simulink model "Sim2Real_ankle_motion_2025a"  (R2025a)
settings: Solver=FixedStepDiscrete  StartTime=0.0  StopTime=8  FixedStep=Ts_1ms  MaxStep=0.002  RelTol=1e-3
InitFcn:
  | modelFile = get_param(bdroot,'FileName');
  | if isempty(modelFile)
  |     error('The model must be saved before running InitFcn.');
  | end
  | 
  | % Folder where the .slx model is located
  | modelFolder = fileparts(char(modelFile));
  | 
  | % Find the parent folder named "resources" by going upwards
  | currentFolder  = modelFolder;
  | materialFolder = '';
  | 
  | while true
  |     [parentFolder, currentName] = fileparts(currentFolder);
  | 
  |     if strcmpi(currentName, 'resources')
  |         materialFolder = currentFolder;
  |         break;
  |     end
  | 
  |     if strcmp(parentFolder, currentFolder)
  |         error('Could not find a parent folder named "resources" starting from: %s', modelFolder);
  |     end
  | 
  |     currentFolder = parentFolder;
  | end
  | 
  | % Search recursively for the MuJoCo XML inside "material"
  | xmlSearch = dir(fullfile(materialFolder, '**', 'unitree_G1.xml'));
  | 
  | if isempty(xmlSearch)
  |     error('MuJoCo XML file not found inside material folder: %s', materialFolder);
  | elseif numel(xmlSearch) > 1
  |     error('Multiple unitree_G1.xml files found inside material folder. Leave only one valid XML.');
  | end
  | 
  | mujocoFolder = xmlSearch(1).folder;
  | xmlFullPath  = fullfile(xmlSearch(1).folder, xmlSearch(1).name);
  | 
  | % Save in base workspace in case you want to inspect them
  | assignin('base','modelFolder',modelFolder);
  | assignin('base','materialFolder',materialFolder);
  | assignin('base','mujocoFolder',mujocoFolder);
  | assignin('base','xmlFullPath',xmlFullPath);
  | 
  | % Final existence check
  | if exist(xmlFullPath,'file') ~= 2
  |     error('MuJoCo XML file not found: %s', xmlFullPath);
  | end
  | 
  | % Add the XML folder to the path so WHICH can find it
  | addpath(mujocoFolder, '-begin');
  | rehash path;
  | 
  | % Run launcher from the same folder as the model
  | launcherFile = fullfile(modelFolder, 'launcher_ankle_motion.mlx');
  | if exist(launcherFile,'file') == 2
  |     run(launcherFile);
  | else
  |     error('Launcher file not found: %s', launcherFile);
  | end
  | 
  | % RUN_MODE:
  | if evalin('base', "exist('RUN_MODE','var')")
  |     tmp = evalin('base','RUN_MODE');
  |     if isa(tmp,'Simulink.Parameter')
  |         RUN_MODE = tmp;
  |     else
  |         RUN_MODE = Simulink.Parameter(tmp);
  |         RUN_MODE.CoderInfo.StorageClass = 'SimulinkGlobal';
  |         assignin('base','RUN_MODE',RUN_MODE);
  |     end
  | else
  |     RUN_MODE = Simulink.Parameter(0);
  |     RUN_MODE.CoderInfo.StorageClass = 'SimulinkGlobal';
  |     assignin('base','RUN_MODE',RUN_MODE);
  | end
StopFcn:
  | drawnow; pause(0.05);
  | 
  | % Stop figures
  | tags = {'G1_IMUState','G1_MotorState'};
  | for k = 1:numel(tags)
  |     delete(findall(0,'Type','uifigure','Tag',tags{k}));
  |     delete(findall(0,'Type','figure' , 'Tag',tags{k}));
  | end
  | 
  | 
  | % Automatic ankle metrics CSV (installed once)
  | addpath(fileparts(get_param('Sim2Real_ankle_motion_2025a', 'FileName')));
  | ankle_motion_csv('save');
undefined symbols (not defined in the file or in its folder): crc, DiscIntNeverNeededParam, mode_machine, mode_pr, motor_cmd, reserve, Ts_1ms
libraries: ros2lib x3, slpidlib x1, mjLib x1
(part 1 of 2)
settings Model: Creator=vmano  LastModifiedBy=Leffer
settings OptimizationCC: ReuseModelBlockBuffer=off
settings ModelReferenceCC: EnableRefExpFcnMdlSchedulingChecks=on
settings SFSimCC: SimTargetLang=C++  SimDLTargetLibrary=mkl-dnn
settings RTWCC: GPUComputeCapability=3.5

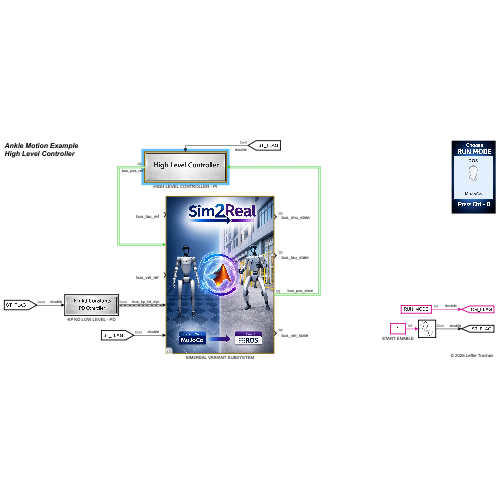
[thumbnail: Simulink's stored preview of the top-level diagram]
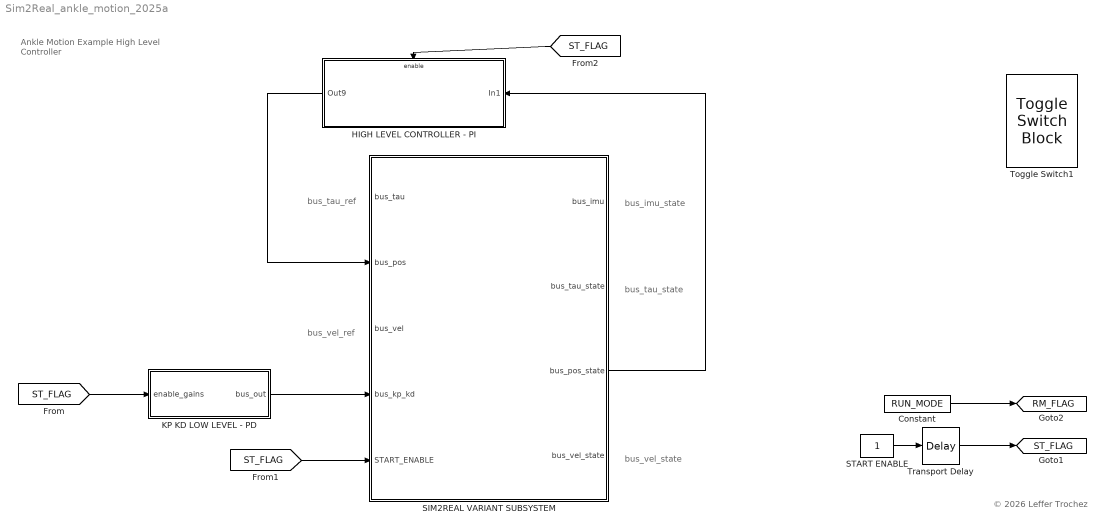
== system Sim2Real_ankle_motion_2025a ==
  note: bus_tau_ref
  note: © 2026 Leffer Trochez
  note: bus_vel_ref
  note: bus_imu_state
  note: bus_tau_state
  note: bus_vel_state
  note: Ankle Motion Example
      | High Level Controller
  Constant : Constant  Value=RUN_MODE
  HIGH LEVEL CONTROLLER - PI : Subsystem  TreatAsAtomicUnit=on
      mask Display: image('16.png');
  KP KD LOW LEVEL - PD : MATLAB Function  TreatAsAtomicUnit=on
  SIM2REAL VARIANT SUBSYSTEM : Subsystem  Variant=on  EmptyChoice=on
      mask Display: image('Sim2RealLogo2.png');
  START ENABLE : Constant
  Toggle Switch1 : ToggleSwitchBlock  LabelPosition=Hide
  Transport Delay : TransportDelay  DelayTime=3  BufferSize=8192
  tag scope: RM_FLAG=global, ST_FLAG=global
  wires:
  Constant/1 -> [RM_FLAG]
  KP KD LOW LEVEL - PD/1(bus_out) -> SIM2REAL VARIANT SUBSYSTEM/4(bus_kp_kd)
  START ENABLE/1 -> Transport Delay/1
  Transport Delay/1 -> [ST_FLAG]
  [ST_FLAG] -> KP KD LOW LEVEL - PD/1(enable_gains)
  [ST_FLAG] -> SIM2REAL VARIANT SUBSYSTEM/5(START_ENABLE)
  SIM2REAL VARIANT SUBSYSTEM/3(bus_pos_state) -> HIGH LEVEL CONTROLLER - PI/1(In1)
  HIGH LEVEL CONTROLLER - PI/1(Out9) -> SIM2REAL VARIANT SUBSYSTEM/2(bus_pos)
  [ST_FLAG] -> HIGH LEVEL CONTROLLER - PI/Enable

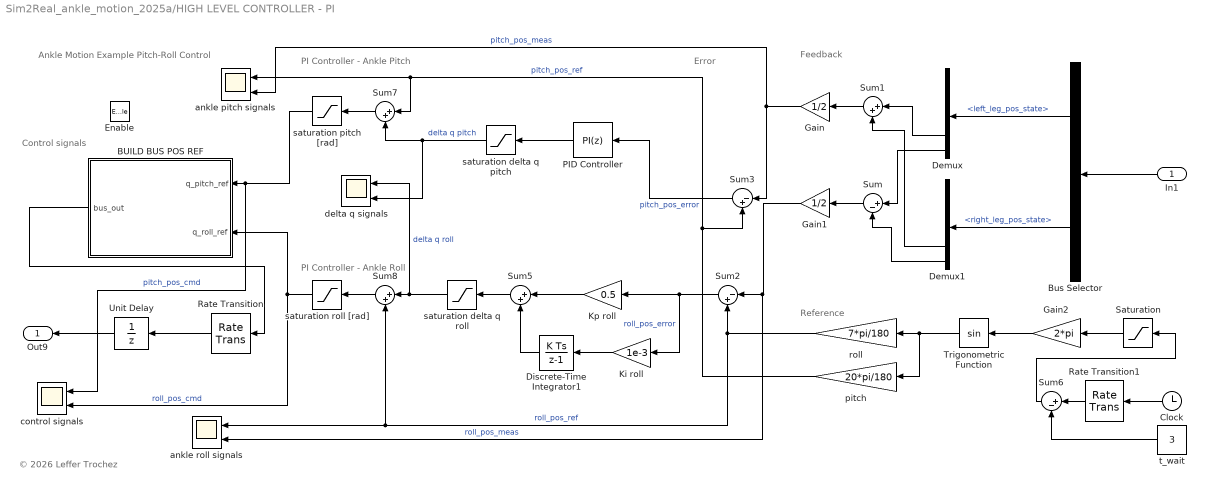
== system Sim2Real_ankle_motion_2025a/HIGH LEVEL CONTROLLER - PI ==
  note: Ankle Motion Example
      | Pitch-Roll Control
  note: Reference
  note: Feedback
  note: PI Controller - Ankle Pitch
  note: PI Controller - Ankle Roll
  note: Error
  note: Control signals
  note: © 2026 Leffer Trochez
  In1 : Inport  OutDataTypeStr=Bus: bus_pos_state
  Enable : EnablePort
  BUILD BUS POS REF : MATLAB Function  TreatAsAtomicUnit=on
  Bus Selector : BusSelector  OutputSignals=left_leg_pos_state,right_leg_pos_state
  Clock : Clock
  Demux : Demux  Outputs=6
  Demux1 : Demux  Outputs=6
  Discrete-Time Integrator1 : DiscreteIntegrator  SampleTime=0.002  ICPrevOutput=DiscIntNeverNeededParam  ICPrevScaledInput=DiscIntNeverNeededParam
  Gain : Gain  Gain=1/2
  Gain1 : Gain  Gain=1/2
  Gain2 : Gain  Gain=2*pi
  Ki roll : Gain  Gain=1e-3
  Kp roll : Gain  Gain=0.5
  "PID Controller " : slpidlib/PID Controller  Controller=PI  Form=Parallel  TimeDomain=Discrete-time  UseExternalTs=off  SampleTime=0.002  IntegratorMethod=Forward Euler  FilterMethod=Forward Euler  ControllerParametersSource=internal  P=0.3  I=0.04  UseKiTs=off  D=0  UseExternalDerivativeSource=off  N=100  UseFilter=on  TunerSelectOption=Transfer Function Based (PID Tuner App)  InitialConditionSource=internal  InitialConditionForIntegrator=0  InitialConditionForFilter=0  DifferentiatorICPrevScaledInput=0  ExternalReset=none  TrackingMode=off  Kt=1  LimitOutput=on  SatLimitsSource=internal  UpperSaturationLimit=0.035  LowerSaturationLimit=-0.035  LinearizeAsGain=on  AntiWindupMode=clamping  Kb=1  LimitIntegrator=off  UpperIntegratorSaturationLimit=inf  LowerIntegratorSaturationLimit=-inf  POutMin=[]  POutMax=[]  IOutMin=[]  IOutMax=[]  DOutMin=[]  DOutMax=[]  NOutMin=[]  NOutMax=[]  SumOutMin=[]  SumOutMax=[]  SaturationOutMin=[]  SaturationOutMax=[]  PParamMin=[]  PParamMax=[]  IParamMin=[]  IParamMax=[]  DParamMin=[]  DParamMax=[]  NParamMin=[]  NParamMax=[]  KbParamMin=[]  KbParamMax=[]  KtParamMin=[]  KtParamMax=[]  KbOutMin=[]  KbOutMax=[]  KtOutMin=[]  KtOutMax=[]  IntegratorOutMin=[]  IntegratorOutMax=[]  FilterOutMin=[]  FilterOutMax=[]  SumI1OutMin=[]  SumI1OutMax=[]  SumI2OutMin=[]  SumI2OutMax=[]  SumI3OutMin=[]  SumI3OutMax=[]  SumI4OutMin=[]  SumI4OutMax=[]  SumDOutMin=[]  SumDOutMax=[]  DifferentiatorOutMin=[]  DifferentiatorOutMax=[]  FilterDiffOutCoefMin=[]  FilterDiffOutCoefMax=[]  ReciprocalOutMin=[]  ReciprocalOutMax=[]  SumDenOutMin=[]  SumDenOutMax=[]  SumNumOutMin=[]  SumNumOutMax=[]  DivideOutMin=[]  DivideOutMax=[]  UdiffTsProdOutMin=[]  UdiffTsProdOutMax=[]  NTsProdOutMin=[]  NTsProdOutMax=[]  UintegralTsProdOutMin=[]  UintegralTsProdOutMax=[]  UngainTsProdOutMin=[]  UngainTsProdOutMax=[]  ClampingZeroOutDataTypeStr=Inherit: Inherit via back propagation  ClampingZeroOutMin=[]  ClampingZeroOutMax=[]  FilterDenConstantOutDataTypeStr=Inherit: Inherit via back propagation  FilterDenConstantOutMin=[]  FilterDenConstantOutMax=[]  PCopyOutDataTypeStr=Inherit: Inherit via back propagation  PCopyOutMin=[]  PCopyOutMax=[]  NCopyOutDataTypeStr=Inherit: Inherit via back propagation  NCopyOutMin=[]  NCopyOutMax=[]  IntegratorContinuousStateAttributes=''  IntegratorStateMustResolveToSignalObject=off  IntegratorRTWStateStorageClass=Auto  FilterContinuousStateAttributes=''  FilterStateMustResolveToSignalObject=off  FilterRTWStateStorageClass=Auto  ParallelPVariant=InternalParameters  IdealPVariant=Disabled  IVariant=InternalParameters  DVariant=Disabled  IntegratorVariant=Discrete  SatVariant=Enabled  AWVariant=DiscClampingParallel  PCopyVariant=Disabled  TRVariant=Disabled  FdbkBlocksVariant=Forward  IdealPFdbkVariant=Disabled  SatFdbkVariant=Disabled  DerivativeFilterVariant=Disabled  NVariant=Disabled  NCopyVariant=Disabled_SignalSpec  FilterICVariant=Disabled  IntegratorICVariant=InternalICs  ExternalResetVariant=Disabled  TRSumVariant=Passthrough  SumFdbkVariant=Disabled  SumVariant=Sum_PI  TsampFilterVariant=InternalTs  TsampNgainVariant=Passthrough  TsampIntegralVariant=Disabled_SignalSpec  ExternalSaturationOutDataTypeStr=Inherit: Same as second input  DerivativeSourceVariant=Disabled  PreIntVariant=InternalPreInt
      settings: LibrarySourceBlock=simulink/Discrete/Discrete PID Controller
  Rate Transition : RateTransition  OutPortSampleTime=Ts_2ms
  Rate Transition1 : RateTransition  OutPortSampleTime=Ts_2ms
  Saturation : Saturate  UpperLimit=inf  LowerLimit=0
  Sum : Sum  Inputs=|+-
  Sum{1,5,7..8} (4 alike) : Sum  Inputs=|++
  Sum2 : Sum  Inputs=|-+
  Sum3 : Sum  Inputs=|-+
  Sum6 : Sum  Inputs=|+-
  Trigonometric Function : Trigonometry
  Unit Delay : UnitDelay  SampleTime=-1  HasFrameUpgradeWarning=on
  ankle pitch signals : Scope  NumInputPorts=2
      settings: Title=Ankle Pitch Signals  ActiveDisplayYMinimum=-0.43633231299858238  ActiveDisplayYMaximum=0.43633231299858238  YLabel=Position [rad]
  ankle roll signals : Scope  NumInputPorts=2
      settings: Title=Ankle Roll Signals  ActiveDisplayYMinimum=-0.15271630954950383  ActiveDisplayYMaximum=0.15271630954950383  YLabel=Position [rad]
  control signals : Scope  NumInputPorts=2
      settings: Title=Torque Position Signals  ActiveDisplayYMinimum=-0.4451715502441761  ActiveDisplayYMaximum=0.44153028177818288  YLabel=Position [rad]  DataLoggingVariableName=ScopeData2
  delta q signals : Scope  NumInputPorts=2
      settings: Title=Delta q Signals  ActiveDisplayYMinimum=-0.0436472558403566  ActiveDisplayYMaximum=0.04282530256320935  DataLoggingVariableName=ScopeData3
  pitch : Gain  Gain=20*pi/180
  roll : Gain  Gain=7*pi/180
  saturation delta q pitch : Saturate  UpperLimit=0.035  LowerLimit=-0.035
  saturation delta q roll : Saturate  UpperLimit=0.025  LowerLimit=-0.025
  saturation pitch [rad] : Saturate  UpperLimit=0.535  LowerLimit=-0.535
  saturation roll [rad] : Saturate  UpperLimit=0.25  LowerLimit=-0.25
  t_wait : Constant  Value=3
  Out9 : Outport  OutDataTypeStr=Bus: bus_pos_ref
  wires:
  Bus Selector/1 -> Demux/1  "<left_leg_pos_state>"
  saturation delta q pitch/1 -> delta q signals/2, Sum7/2  "delta q pitch"
  Gain2/1 -> Trigonometric Function/1
  Rate Transition/1 -> Unit Delay/1
  Sum/1 -> Gain1/1
  "PID Controller "/1 -> saturation delta q pitch/1
  Unit Delay/1 -> Out9/1
  Demux1/6 -> Sum/2
  Kp roll/1 -> Sum5/1
  Sum1/1 -> Gain/1
  Demux1/5 -> Sum1/2
  Discrete-Time Integrator1/1 -> Sum5/2
  Bus Selector/2 -> Demux1/1  "<right_leg_pos_state>"
  Gain1/1 -> ankle roll signals/2, Sum2/1  "roll_pos_meas"
  pitch/1 -> Sum3/2, ankle pitch signals/1, Sum7/1  "pitch_pos_ref"
  Sum3/1 -> "PID Controller "/1  "pitch_pos_error"
  Gain/1 -> ankle pitch signals/2, Sum3/1  "pitch_pos_meas"
  Trigonometric Function/1 -> pitch/1, roll/1
  Ki roll/1 -> Discrete-Time Integrator1/1
  Demux/6 -> Sum/1
  In1/1 -> Bus Selector/1
  Sum2/1 -> Kp roll/1, Ki roll/1  "roll_pos_error"
  Demux/5 -> Sum1/1
  BUILD BUS POS REF/1(bus_out) -> Rate Transition/1
  Clock/1 -> Rate Transition1/1
  Sum6/1 -> Saturation/1
  t_wait/1 -> Sum6/2
  Saturation/1 -> Gain2/1
  Rate Transition1/1 -> Sum6/1
  Sum7/1 -> saturation pitch [rad]/1
  saturation pitch [rad]/1 -> control signals/1, BUILD BUS POS REF/1(q_pitch_ref)  "pitch_pos_cmd"
  Sum8/1 -> saturation roll [rad]/1
  saturation delta q roll/1 -> delta q signals/1, Sum8/1  "delta q roll"
  Sum5/1 -> saturation delta q roll/1
  roll/1 -> Sum8/2, ankle roll signals/1, Sum2/2  "roll_pos_ref"
  saturation roll [rad]/1 -> control signals/2, BUILD BUS POS REF/2(q_roll_ref)  "roll_pos_cmd"

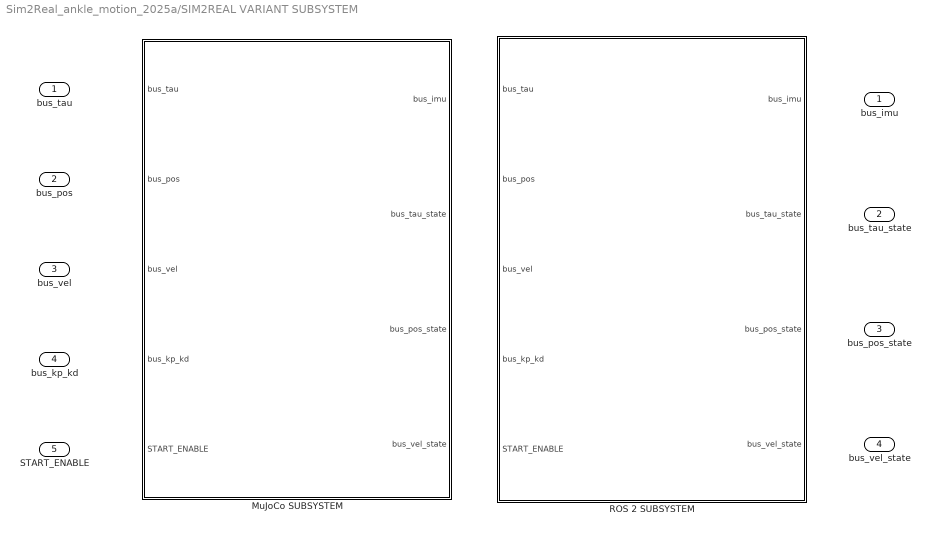
== system Sim2Real_ankle_motion_2025a/SIM2REAL VARIANT SUBSYSTEM ==
  bus_tau : Inport  OutDataTypeStr=Bus: bus_tau_ref
  bus_pos : Inport  Port=2  OutDataTypeStr=Bus: bus_pos_ref
  bus_vel : Inport  Port=3  OutDataTypeStr=Bus: bus_vel_ref
  bus_kp_kd : Inport  Port=4  OutDataTypeStr=Bus: bus_kp_kd_dyn
  START_ENABLE : Inport  Port=5
  MuJoCo SUBSYSTEM : Subsystem  VariantControl=RUN_MODE == 0
      mask Display: image('MuJoCo G1.png');
  ROS 2 SUBSYSTEM : Subsystem  VariantControl=RUN_MODE == 1
      mask Display: image('Real G1.png');
  bus_imu : Outport  OutDataTypeStr=Bus: bus_imu
  bus_tau_state : Outport  Port=2  OutDataTypeStr=Bus: bus_tau_state
  bus_pos_state : Outport  Port=3  OutDataTypeStr=Bus: bus_pos_state
  bus_vel_state : Outport  Port=4  OutDataTypeStr=Bus: bus_vel_state

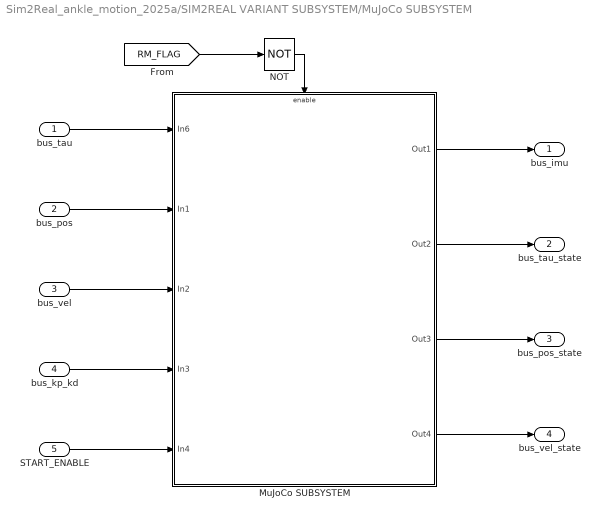
== system Sim2Real_ankle_motion_2025a/SIM2REAL VARIANT SUBSYSTEM/MuJoCo SUBSYSTEM ==
  bus_tau : Inport  OutDataTypeStr=Bus: bus_tau_ref
  bus_pos : Inport  Port=2  OutDataTypeStr=Bus: bus_pos_ref
  bus_vel : Inport  Port=3  OutDataTypeStr=Bus: bus_vel_ref
  bus_kp_kd : Inport  Port=4  OutDataTypeStr=Bus: bus_kp_kd_dyn
  START_ENABLE : Inport  Port=5
  MuJoCo SUBSYSTEM : Subsystem  TreatAsAtomicUnit=on
      mask Display: image('MuJoCo G1.png');
  NOT : Logic  Operator=NOT  IconShape=distinctive  AllPortsSameDT=off  OutDataTypeStr=boolean
  bus_imu : Outport  OutDataTypeStr=Bus: bus_imu
  bus_tau_state : Outport  Port=2  OutDataTypeStr=Bus: bus_tau_state
  bus_pos_state : Outport  Port=3  OutDataTypeStr=Bus: bus_pos_state
  bus_vel_state : Outport  Port=4  OutDataTypeStr=Bus: bus_vel_state
  wires:
  [RM_FLAG] -> NOT/1
  NOT/1 -> MuJoCo SUBSYSTEM/Enable
  bus_tau/1 -> MuJoCo SUBSYSTEM/1(In6)
  bus_pos/1 -> MuJoCo SUBSYSTEM/2(In1)
  bus_vel/1 -> MuJoCo SUBSYSTEM/3(In2)
  bus_kp_kd/1 -> MuJoCo SUBSYSTEM/4(In3)
  START_ENABLE/1 -> MuJoCo SUBSYSTEM/5(In4)
  MuJoCo SUBSYSTEM/1(Out1) -> bus_imu/1
  MuJoCo SUBSYSTEM/2(Out2) -> bus_tau_state/1
  MuJoCo SUBSYSTEM/3(Out3) -> bus_pos_state/1
  MuJoCo SUBSYSTEM/4(Out4) -> bus_vel_state/1

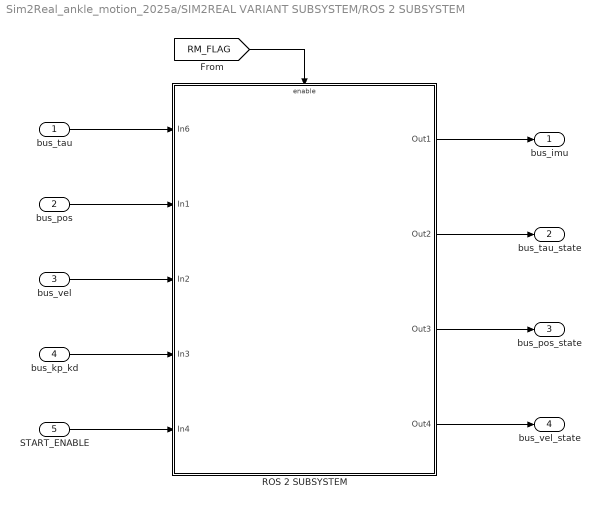
== system Sim2Real_ankle_motion_2025a/SIM2REAL VARIANT SUBSYSTEM/ROS 2 SUBSYSTEM ==
  bus_tau : Inport  OutDataTypeStr=Bus: bus_tau_ref
  bus_pos : Inport  Port=2  OutDataTypeStr=Bus: bus_pos_ref
  bus_vel : Inport  Port=3  OutDataTypeStr=Bus: bus_vel_ref
  bus_kp_kd : Inport  Port=4  OutDataTypeStr=Bus: bus_kp_kd_dyn
  START_ENABLE : Inport  Port=5
  ROS 2 SUBSYSTEM : Subsystem  TreatAsAtomicUnit=on
      mask Display: image('Real G1.png');
  bus_imu : Outport  OutDataTypeStr=Bus: bus_imu
  bus_tau_state : Outport  Port=2  OutDataTypeStr=Bus: bus_tau_state
  bus_pos_state : Outport  Port=3  OutDataTypeStr=Bus: bus_pos_state
  bus_vel_state : Outport  Port=4  OutDataTypeStr=Bus: bus_vel_state
  wires:
  bus_tau/1 -> ROS 2 SUBSYSTEM/1(In6)
  bus_kp_kd/1 -> ROS 2 SUBSYSTEM/4(In3)
  bus_vel/1 -> ROS 2 SUBSYSTEM/3(In2)
  START_ENABLE/1 -> ROS 2 SUBSYSTEM/5(In4)
  bus_pos/1 -> ROS 2 SUBSYSTEM/2(In1)
  ROS 2 SUBSYSTEM/3(Out3) -> bus_pos_state/1
  ROS 2 SUBSYSTEM/2(Out2) -> bus_tau_state/1
  ROS 2 SUBSYSTEM/1(Out1) -> bus_imu/1
  ROS 2 SUBSYSTEM/4(Out4) -> bus_vel_state/1
  [RM_FLAG] -> ROS 2 SUBSYSTEM/Enable

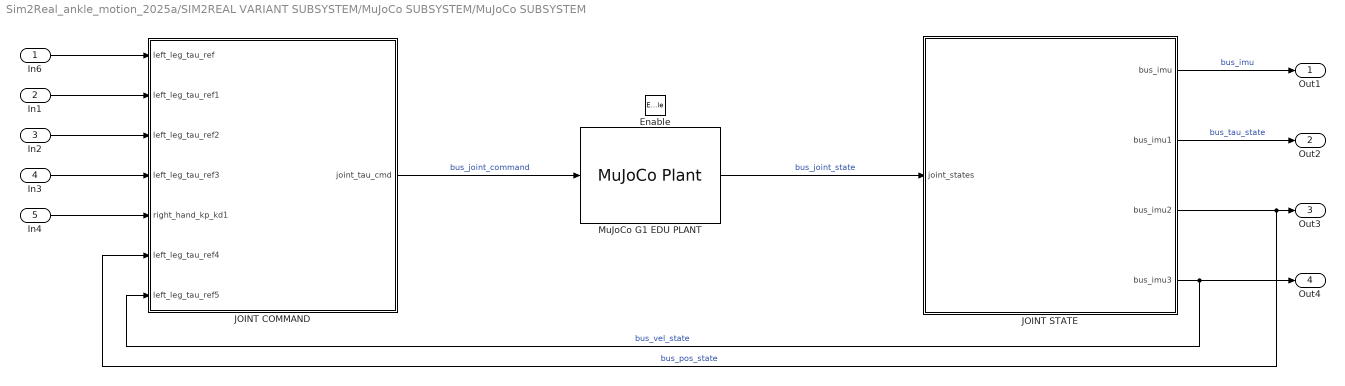
== system Sim2Real_ankle_motion_2025a/SIM2REAL VARIANT SUBSYSTEM/MuJoCo SUBSYSTEM/MuJoCo SUBSYSTEM ==
  In6 : Inport  OutDataTypeStr=Bus: bus_tau_ref
  In1 : Inport  Port=2  OutDataTypeStr=Bus: bus_pos_ref
  In2 : Inport  Port=3  OutDataTypeStr=Bus: bus_vel_ref
  In3 : Inport  Port=4  OutDataTypeStr=Bus: bus_kp_kd_dyn
  In4 : Inport  Port=5
  Enable : EnablePort
  JOINT COMMAND : Subsystem
      mask Display: image('1.png');
  JOINT STATE : Subsystem
      mask Display: image('2.png');
  MuJoCo G1 EDU PLANT : mjLib/MuJoCo Plant  controlBus=[]  sensorBus=mj_bus_sensor_7979902499018342666  controlLength=[]  sensorLength=[]  rgbLength=[]  depthLength=[]  sampleTime=0.002  xmlFileRel=unitree_G1.xml  xmlFile=C:\Users\Leffer\Downloads\resources\MuJoCo files\unitree_G1.xml  renderingType=Global  vsync=off  visualFPS=FPS_MuJoCo  zoomLevel=1  znear=0.032  zfar=160  cameraSampleTime=Ts_1ms  rgbOutOption=on  depthOutOption=off  controlInterfaceType=Bus
      settings: SourceProductName=MuJoCo Simulator
  Out1 : Outport  OutDataTypeStr=Bus: bus_imu
  Out2 : Outport  Port=2  OutDataTypeStr=Bus: bus_tau_state
  Out3 : Outport  Port=3  OutDataTypeStr=Bus: bus_pos_state
  Out4 : Outport  Port=4  OutDataTypeStr=Bus: bus_vel_state
  wires:
  JOINT COMMAND/1(joint_tau_cmd) -> MuJoCo G1 EDU PLANT/1  "bus_joint_command"
  MuJoCo G1 EDU PLANT/1 -> JOINT STATE/1(joint_states)  "bus_joint_state"
  In6/1 -> JOINT COMMAND/1(left_leg_tau_ref)
  In1/1 -> JOINT COMMAND/2(left_leg_tau_ref1)
  In2/1 -> JOINT COMMAND/3(left_leg_tau_ref2)
  In3/1 -> JOINT COMMAND/4(left_leg_tau_ref3)
  In4/1 -> JOINT COMMAND/5(right_hand_kp_kd1)
  JOINT STATE/2(bus_imu1) -> Out2/1  "bus_tau_state"
  JOINT STATE/3(bus_imu2) -> JOINT COMMAND/6(left_leg_tau_ref4), Out3/1  "bus_pos_state"
  JOINT STATE/4(bus_imu3) -> Out4/1, JOINT COMMAND/7(left_leg_tau_ref5)  "bus_vel_state"
  JOINT STATE/1(bus_imu) -> Out1/1  "bus_imu"

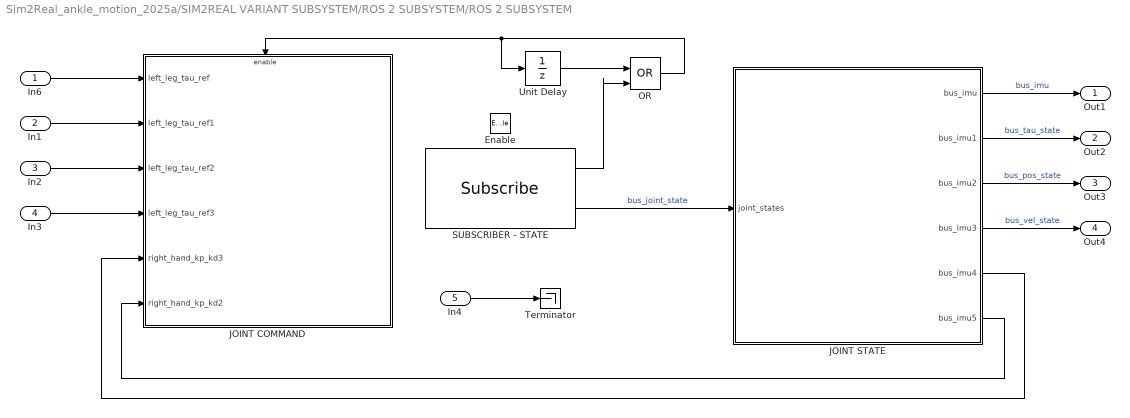
== system Sim2Real_ankle_motion_2025a/SIM2REAL VARIANT SUBSYSTEM/ROS 2 SUBSYSTEM/ROS 2 SUBSYSTEM ==
  In6 : Inport  OutDataTypeStr=Bus: bus_tau_ref
  In1 : Inport  Port=2  OutDataTypeStr=Bus: bus_pos_ref
  In2 : Inport  Port=3  OutDataTypeStr=Bus: bus_vel_ref
  In3 : Inport  Port=4  OutDataTypeStr=Bus: bus_kp_kd_dyn
  In4 : Inport  Port=5
  Enable : EnablePort
  JOINT COMMAND : Subsystem  TreatAsAtomicUnit=on
      mask Display: image('8.png');
  JOINT STATE : Subsystem
      mask Display: image('9.png');
  OR : Logic  Operator=OR  IconShape=distinctive  AllPortsSameDT=off  OutDataTypeStr=boolean
  SUBSCRIBER - STATE : ros2lib/Subscribe  topicSource=Specify your own  topic=/lowstate  messageType=unitree_hg/LowState  sampleTime=Ts_1ms  QOSHistory=Keep last  QOSDepth=10  QOSReliability=Reliable  QOSDurability=Volatile  QOSDeadline=Inf  QOSLifespan=Inf  QOSLiveliness=Automatic  QOSLeaseDuration=Inf  QOSAvoidROSNamespaceConventions=off
  Terminator : Terminator
  Unit Delay : UnitDelay  SampleTime=0.002  HasFrameUpgradeWarning=on
  Out1 : Outport  OutDataTypeStr=Bus: bus_imu
  Out2 : Outport  Port=2  OutDataTypeStr=Bus: bus_tau_state
  Out3 : Outport  Port=3  OutDataTypeStr=Bus: bus_pos_state
  Out4 : Outport  Port=4  OutDataTypeStr=Bus: bus_vel_state
  wires:
  SUBSCRIBER - STATE/2 -> JOINT STATE/1(joint_states)  "bus_joint_state"
  SUBSCRIBER - STATE/1 -> OR/2
  OR/1 -> JOINT COMMAND/Enable, Unit Delay/1
  Unit Delay/1 -> OR/1
  JOINT STATE/6(bus_imu5) -> JOINT COMMAND/6(right_hand_kp_kd2)
  In2/1 -> JOINT COMMAND/3(left_leg_tau_ref2)
  In3/1 -> JOINT COMMAND/4(left_leg_tau_ref3)
  In4/1 -> Terminator/1
  In1/1 -> JOINT COMMAND/2(left_leg_tau_ref1)
  In6/1 -> JOINT COMMAND/1(left_leg_tau_ref)
  JOINT STATE/4(bus_imu3) -> Out4/1  "bus_vel_state"
  JOINT STATE/3(bus_imu2) -> Out3/1  "bus_pos_state"
  JOINT STATE/2(bus_imu1) -> Out2/1  "bus_tau_state"
  JOINT STATE/1(bus_imu) -> Out1/1  "bus_imu"
  JOINT STATE/5(bus_imu4) -> JOINT COMMAND/5(right_hand_kp_kd3)

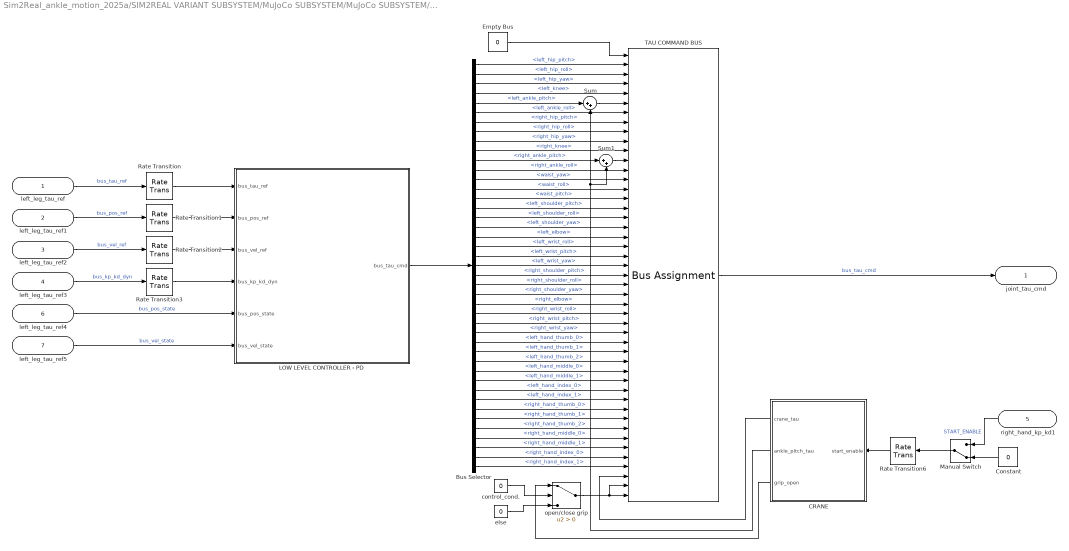
== system Sim2Real_ankle_motion_2025a/SIM2REAL VARIANT SUBSYSTEM/MuJoCo SUBSYSTEM/MuJoCo SUBSYSTEM/JOINT COMMAND ==
  left_leg_tau_ref : Inport  OutDataTypeStr=Bus: bus_tau_ref
  left_leg_tau_ref1 : Inport  Port=2  OutDataTypeStr=Bus: bus_pos_ref
  left_leg_tau_ref2 : Inport  Port=3  OutDataTypeStr=Bus: bus_vel_ref
  left_leg_tau_ref3 : Inport  Port=4  OutDataTypeStr=Bus: bus_kp_kd_dyn
  right_hand_kp_kd1 : Inport  Port=5
  left_leg_tau_ref4 : Inport  Port=6  OutDataTypeStr=Bus: bus_pos_state
  left_leg_tau_ref5 : Inport  Port=7  OutDataTypeStr=Bus: bus_vel_state
  Bus Selector : BusSelector  OutputSignals=left_hip_pitch,left_hip_roll,left_hip_yaw,left_knee,left_ankle_pitch,left_ankle_roll,right_hip_pitch,right_hip_roll,right_hip_yaw,right_knee,right_ankle_pitch,right_ankle_roll,waist_yaw,waist_roll,waist_pitch,left_shoulder_pitch,left_shoulder_roll,left_shoulder_yaw,left_elbow,left_wrist_roll,left_wrist_pitch,left_wrist_yaw,right_shoulder_pitch,right_shoulder_roll,right_shoulder_yaw,right_elbow,right_wrist_roll,right_wrist_pitch,right_wrist_yaw,left_hand_thumb_0,left_hand_thumb_1,left_hand_thumb_2,left_hand_middle_0,left_hand_middle_1,left_hand_index_0,left_hand_index_1,right_hand_thumb_0,right_hand_thumb_1,right_hand_thumb_2,right_hand_middle_0,right_hand_middle_1,right_hand_index_0,right_hand_index_1
  CRANE : MATLAB Function  TreatAsAtomicUnit=on
  Constant : Constant  Value=0
  Empty Bus : Constant  Value=0  OutDataTypeStr=Bus: mj_bus_input_303657145477151593  LockScale=on
  LOW LEVEL CONTROLLER - PD : MATLAB Function  TreatAsAtomicUnit=on
  Manual Switch : ManualSwitch  CurrentSetting=0
  Rate Transition{,1..3,6} (5 alike) : RateTransition  OutPortSampleTime=Ts_1ms
  Sum : Sum  Inputs=|++
  Sum1 : Sum  Inputs=|++
  TAU COMMAND BUS : BusAssignment  AssignedSignals=left_hip_pitch,left_hip_roll,left_hip_yaw,left_knee,left_ankle_pitch,left_ankle_roll,right_hip_pitch,right_hip_roll,right_hip_yaw,right_knee,right_ankle_pitch,right_ankle_roll,waist_yaw,waist_roll,waist_pitch,left_shoulder_pitch,left_shoulder_roll,left_shoulder_yaw,left_elbow,left_wrist_roll,left_wrist_pitch,left_wrist_yaw,right_shoulder_pitch,right_shoulder_roll,right_shoulder_yaw,right_elbow,right_wrist_roll,right_wrist_pitch,right_wrist_yaw,left_hand_thumb_0,left_hand_thumb_1,left_hand_thumb_2,left_hand_middle_0,left_hand_middle_1,left_hand_index_0,left_hand_index_1,right_hand_thumb_0,right_hand_thumb_1,right_hand_thumb_2,right_hand_middle_0,right_hand_middle_1,right_hand_index_0,right_hand_index_1,crane_tau,grip_open_R,grip_open_L
  control_cond. : Constant  Value=0
  else : Constant  Value=0
  open/close grip : Switch  Criteria=u2 > Threshold  SaturateOnIntegerOverflow=off  InputSameDT=off
  joint_tau_cmd : Outport  OutDataTypeStr=Bus: mj_bus_input_303657145477151593
  wires:
  Sum1/1 -> TAU COMMAND BUS/12
  Empty Bus/1 -> TAU COMMAND BUS/1
  CRANE/2(ankle_pitch_tau) -> Sum1/2, Sum/2
  Sum/1 -> TAU COMMAND BUS/6
  CRANE/3(grip_open) -> open/close grip/1
  right_hand_kp_kd1/1 -> Manual Switch/1  "START_ENABLE"
  TAU COMMAND BUS/1 -> joint_tau_cmd/1  "bus_tau_cmd"
  left_leg_tau_ref/1 -> Rate Transition/1  "bus_tau_ref"
  left_leg_tau_ref1/1 -> Rate Transition1/1  "bus_pos_ref"
  left_leg_tau_ref2/1 -> Rate Transition2/1  "bus_vel_ref"
  left_leg_tau_ref3/1 -> Rate Transition3/1  "bus_kp_kd_dyn"
  left_leg_tau_ref4/1 -> LOW LEVEL CONTROLLER - PD/5(bus_pos_state)  "bus_pos_state"
  left_leg_tau_ref5/1 -> LOW LEVEL CONTROLLER - PD/6(bus_vel_state)  "bus_vel_state"
  CRANE/1(crane_tau) -> TAU COMMAND BUS/45
  Rate Transition/1 -> LOW LEVEL CONTROLLER - PD/1(bus_tau_ref)
  Rate Transition1/1 -> LOW LEVEL CONTROLLER - PD/2(bus_pos_ref)
  Rate Transition2/1 -> LOW LEVEL CONTROLLER - PD/3(bus_vel_ref)
  Rate Transition3/1 -> LOW LEVEL CONTROLLER - PD/4(bus_kp_kd_dyn)
  Rate Transition6/1 -> CRANE/1(start_enable)
  LOW LEVEL CONTROLLER - PD/1(bus_tau_cmd) -> Bus Selector/1
  Bus Selector/11 -> Sum1/1  "<right_ankle_pitch>"
  Bus Selector/5 -> Sum/1  "<left_ankle_pitch>"
  Bus Selector/1 -> TAU COMMAND BUS/2  "<left_hip_pitch>"
  Bus Selector/2 -> TAU COMMAND BUS/3  "<left_hip_roll>"
  Bus Selector/3 -> TAU COMMAND BUS/4  "<left_hip_yaw>"
  Bus Selector/4 -> TAU COMMAND BUS/5  "<left_knee>"
  Bus Selector/6 -> TAU COMMAND BUS/7  "<left_ankle_roll>"
  Bus Selector/7 -> TAU COMMAND BUS/8  "<right_hip_pitch>"
  Bus Selector/8 -> TAU COMMAND BUS/9  "<right_hip_roll>"
  Bus Selector/9 -> TAU COMMAND BUS/10  "<right_hip_yaw>"
  Bus Selector/10 -> TAU COMMAND BUS/11  "<right_knee>"
  Bus Selector/12 -> TAU COMMAND BUS/13  "<right_ankle_roll>"
  Bus Selector/13 -> TAU COMMAND BUS/14  "<waist_yaw>"
  Bus Selector/14 -> TAU COMMAND BUS/15  "<waist_roll>"
  Bus Selector/15 -> TAU COMMAND BUS/16  "<waist_pitch>"
  Bus Selector/16 -> TAU COMMAND BUS/17  "<left_shoulder_pitch>"
  Bus Selector/17 -> TAU COMMAND BUS/18  "<left_shoulder_roll>"
  Bus Selector/18 -> TAU COMMAND BUS/19  "<left_shoulder_yaw>"
  Bus Selector/19 -> TAU COMMAND BUS/20  "<left_elbow>"
  Bus Selector/20 -> TAU COMMAND BUS/21  "<left_wrist_roll>"
  Bus Selector/21 -> TAU COMMAND BUS/22  "<left_wrist_pitch>"
  Bus Selector/22 -> TAU COMMAND BUS/23  "<left_wrist_yaw>"
  Bus Selector/23 -> TAU COMMAND BUS/24  "<right_shoulder_pitch>"
  Bus Selector/24 -> TAU COMMAND BUS/25  "<right_shoulder_roll>"
  Bus Selector/25 -> TAU COMMAND BUS/26  "<right_shoulder_yaw>"
  Bus Selector/26 -> TAU COMMAND BUS/27  "<right_elbow>"
  Bus Selector/27 -> TAU COMMAND BUS/28  "<right_wrist_roll>"
  Bus Selector/28 -> TAU COMMAND BUS/29  "<right_wrist_pitch>"
  Bus Selector/29 -> TAU COMMAND BUS/30  "<right_wrist_yaw>"
  Bus Selector/30 -> TAU COMMAND BUS/31  "<left_hand_thumb_0>"
  Bus Selector/31 -> TAU COMMAND BUS/32  "<left_hand_thumb_1>"
  Bus Selector/32 -> TAU COMMAND BUS/33  "<left_hand_thumb_2>"
  Bus Selector/33 -> TAU COMMAND BUS/34  "<left_hand_middle_0>"
  Bus Selector/34 -> TAU COMMAND BUS/35  "<left_hand_middle_1>"
  Bus Selector/35 -> TAU COMMAND BUS/36  "<left_hand_index_0>"
  Bus Selector/36 -> TAU COMMAND BUS/37  "<left_hand_index_1>"
  Bus Selector/37 -> TAU COMMAND BUS/38  "<right_hand_thumb_0>"
  Bus Selector/38 -> TAU COMMAND BUS/39  "<right_hand_thumb_1>"
  Bus Selector/39 -> TAU COMMAND BUS/40  "<right_hand_thumb_2>"
  Bus Selector/40 -> TAU COMMAND BUS/41  "<right_hand_middle_0>"
  Bus Selector/41 -> TAU COMMAND BUS/42  "<right_hand_middle_1>"
  Bus Selector/42 -> TAU COMMAND BUS/43  "<right_hand_index_0>"
  Bus Selector/43 -> TAU COMMAND BUS/44  "<right_hand_index_1>"
  control_cond./1 -> open/close grip/2
  else/1 -> open/close grip/3
  open/close grip/1 -> TAU COMMAND BUS/47, TAU COMMAND BUS/46
  Manual Switch/1 -> Rate Transition6/1
  Constant/1 -> Manual Switch/2

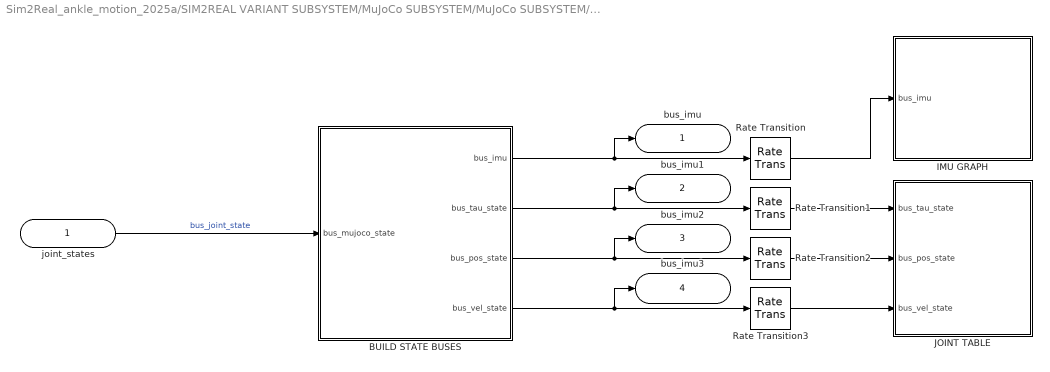
== system Sim2Real_ankle_motion_2025a/SIM2REAL VARIANT SUBSYSTEM/MuJoCo SUBSYSTEM/MuJoCo SUBSYSTEM/JOINT STATE ==
  joint_states : Inport  OutDataTypeStr=Bus: mj_bus_sensor_13323796724550544295
  BUILD STATE BUSES : MATLAB Function  TreatAsAtomicUnit=on
  IMU GRAPH : MATLAB Function  TreatAsAtomicUnit=on
  JOINT TABLE : MATLAB Function  TreatAsAtomicUnit=on
  Rate Transition{,1..3} (4 alike) : RateTransition  OutPortSampleTime=Ts_UIs
  bus_imu : Outport  OutDataTypeStr=Bus: bus_imu
  bus_imu1 : Outport  Port=2  OutDataTypeStr=Bus: bus_tau_state
  bus_imu2 : Outport  Port=3  OutDataTypeStr=Bus: bus_pos_state
  bus_imu3 : Outport  Port=4  OutDataTypeStr=Bus: bus_vel_state
  wires:
  joint_states/1 -> BUILD STATE BUSES/1(bus_mujoco_state)  "bus_joint_state"
  BUILD STATE BUSES/1(bus_imu) -> Rate Transition/1, bus_imu/1
  BUILD STATE BUSES/3(bus_pos_state) -> Rate Transition2/1, bus_imu2/1
  BUILD STATE BUSES/2(bus_tau_state) -> Rate Transition1/1, bus_imu1/1
  BUILD STATE BUSES/4(bus_vel_state) -> Rate Transition3/1, bus_imu3/1
  Rate Transition/1 -> IMU GRAPH/1(bus_imu)
  Rate Transition1/1 -> JOINT TABLE/1(bus_tau_state)
  Rate Transition2/1 -> JOINT TABLE/2(bus_pos_state)
  Rate Transition3/1 -> JOINT TABLE/3(bus_vel_state)

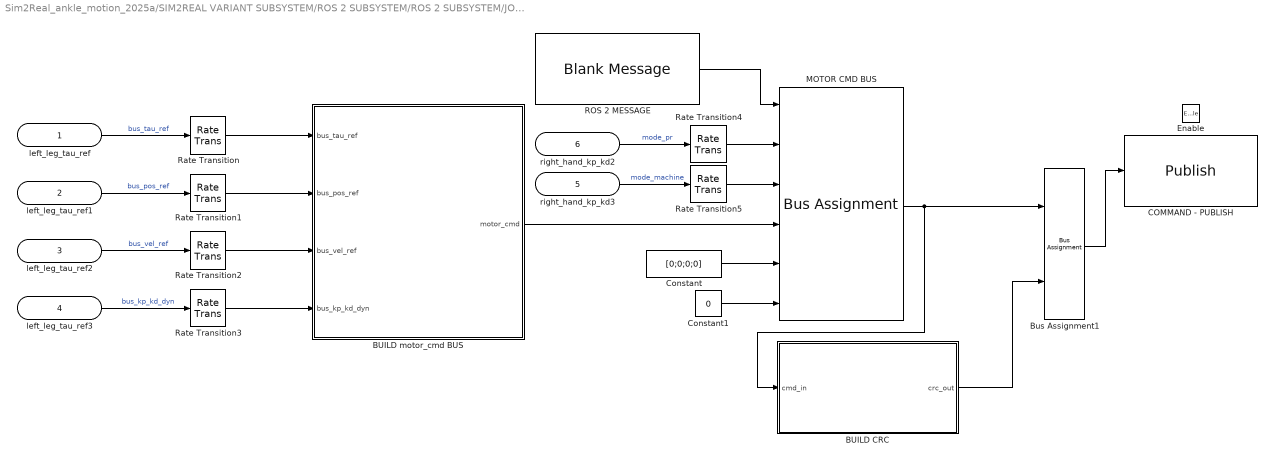
== system Sim2Real_ankle_motion_2025a/SIM2REAL VARIANT SUBSYSTEM/ROS 2 SUBSYSTEM/ROS 2 SUBSYSTEM/JOINT COMMAND ==
  left_leg_tau_ref : Inport  OutDataTypeStr=Bus: bus_tau_ref
  left_leg_tau_ref1 : Inport  Port=2  OutDataTypeStr=Bus: bus_pos_ref
  left_leg_tau_ref2 : Inport  Port=3  OutDataTypeStr=Bus: bus_vel_ref
  left_leg_tau_ref3 : Inport  Port=4  OutDataTypeStr=Bus: bus_kp_kd_dyn
  right_hand_kp_kd3 : Inport  Port=5
  right_hand_kp_kd2 : Inport  Port=6
  Enable : EnablePort
  BUILD CRC : MATLAB Function  TreatAsAtomicUnit=on
  BUILD motor_cmd BUS : MATLAB Function  TreatAsAtomicUnit=on
  Bus Assignment1 : BusAssignment  AssignedSignals=crc
  COMMAND - PUBLISH : ros2lib/Publish  topicSource=Specify your own  topic=/lowcmd  messageType=unitree_hg/LowCmd  QOSHistory=Keep last  QOSDepth=10  QOSReliability=Reliable  QOSDurability=Volatile  QOSDeadline=Inf  QOSLifespan=Inf  QOSLiveliness=Automatic  QOSLeaseDuration=Inf  QOSAvoidROSNamespaceConventions=off
  Constant : Constant  Value=[0;0;0;0]  OutDataTypeStr=uint32
  Constant1 : Constant  Value=0  OutDataTypeStr=uint32
  MOTOR CMD BUS : BusAssignment  AssignedSignals=mode_pr,mode_machine,motor_cmd,reserve,crc
  ROS 2 MESSAGE : ros2lib/Blank Message  messageClass=Message  entityType=unitree_hg/LowCmd  messageType=unitree_hg/LowCmd  SampleTime=Ts_1ms
  Rate Transition{,1..5} (6 alike) : RateTransition  OutPortSampleTime=Ts_1ms
  wires:
  right_hand_kp_kd3/1 -> Rate Transition5/1  "mode_machine"
  left_leg_tau_ref/1 -> Rate Transition/1  "bus_tau_ref"
  right_hand_kp_kd2/1 -> Rate Transition4/1  "mode_pr"
  ROS 2 MESSAGE/1 -> MOTOR CMD BUS/1
  BUILD motor_cmd BUS/1(motor_cmd) -> MOTOR CMD BUS/4
  MOTOR CMD BUS/1 -> BUILD CRC/1(cmd_in), Bus Assignment1/1
  BUILD CRC/1(crc_out) -> Bus Assignment1/2
  Constant/1 -> MOTOR CMD BUS/5
  Constant1/1 -> MOTOR CMD BUS/6
  Bus Assignment1/1 -> COMMAND - PUBLISH/1
  left_leg_tau_ref1/1 -> Rate Transition1/1  "bus_pos_ref"
  left_leg_tau_ref2/1 -> Rate Transition2/1  "bus_vel_ref"
  left_leg_tau_ref3/1 -> Rate Transition3/1  "bus_kp_kd_dyn"
  Rate Transition/1 -> BUILD motor_cmd BUS/1(bus_tau_ref)
  Rate Transition1/1 -> BUILD motor_cmd BUS/2(bus_pos_ref)
  Rate Transition2/1 -> BUILD motor_cmd BUS/3(bus_vel_ref)
  Rate Transition3/1 -> BUILD motor_cmd BUS/4(bus_kp_kd_dyn)
  Rate Transition4/1 -> MOTOR CMD BUS/2
  Rate Transition5/1 -> MOTOR CMD BUS/3

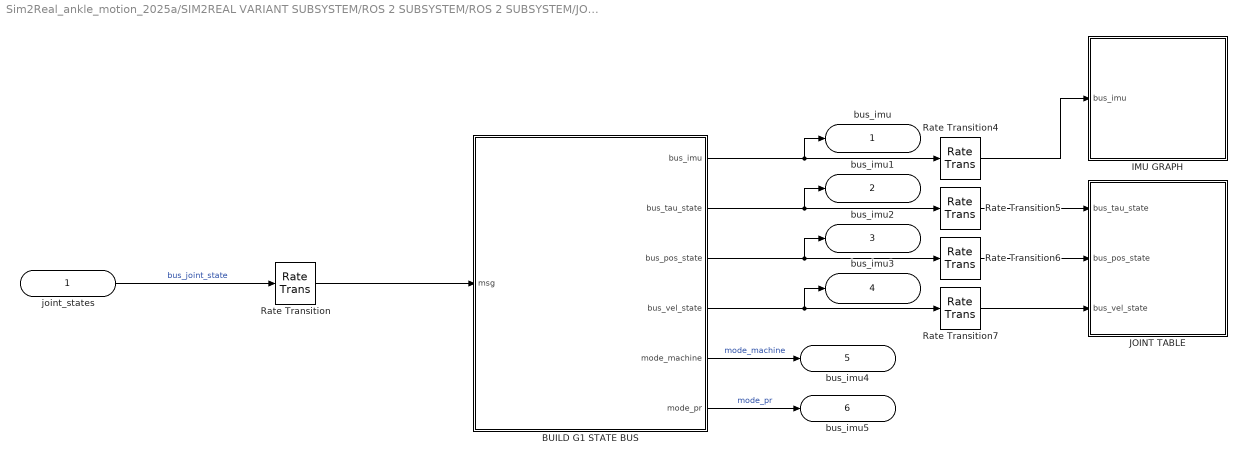
== system Sim2Real_ankle_motion_2025a/SIM2REAL VARIANT SUBSYSTEM/ROS 2 SUBSYSTEM/ROS 2 SUBSYSTEM/JOINT STATE ==
  joint_states : Inport
  BUILD G1 STATE BUS : MATLAB Function  TreatAsAtomicUnit=on
  IMU GRAPH : MATLAB Function  TreatAsAtomicUnit=on
  JOINT TABLE : MATLAB Function  TreatAsAtomicUnit=on
  Rate Transition : RateTransition  OutPortSampleTime=0.002
  Rate Transition{4..7} (4 alike) : RateTransition  OutPortSampleTime=Ts_UIs
  bus_imu : Outport  OutDataTypeStr=Bus: bus_imu
  bus_imu1 : Outport  Port=2  OutDataTypeStr=Bus: bus_tau_state
  bus_imu2 : Outport  Port=3  OutDataTypeStr=Bus: bus_pos_state
  bus_imu3 : Outport  Port=4  OutDataTypeStr=Bus: bus_vel_state
  bus_imu4 : Outport  Port=5
  bus_imu5 : Outport  Port=6
  wires:
  joint_states/1 -> Rate Transition/1  "bus_joint_state"
  BUILD G1 STATE BUS/5(mode_machine) -> bus_imu4/1  "mode_machine"
  BUILD G1 STATE BUS/6(mode_pr) -> bus_imu5/1  "mode_pr"
  Rate Transition5/1 -> JOINT TABLE/1(bus_tau_state)
  Rate Transition6/1 -> JOINT TABLE/2(bus_pos_state)
  BUILD G1 STATE BUS/3(bus_pos_state) -> bus_imu2/1, Rate Transition6/1
  BUILD G1 STATE BUS/2(bus_tau_state) -> bus_imu1/1, Rate Transition5/1
  Rate Transition4/1 -> IMU GRAPH/1(bus_imu)
  BUILD G1 STATE BUS/1(bus_imu) -> bus_imu/1, Rate Transition4/1
  BUILD G1 STATE BUS/4(bus_vel_state) -> bus_imu3/1, Rate Transition7/1
  Rate Transition7/1 -> JOINT TABLE/3(bus_vel_state)
  Rate Transition/1 -> BUILD G1 STATE BUS/1(msg)

== matlab function Sim2Real_ankle_motion_2025a/SIM2REAL VARIANT SUBSYSTEM/MuJoCo SUBSYSTEM/MuJoCo SUBSYSTEM/JOINT COMMAND/LOW LEVEL CONTROLLER - PD ==
  data: bus_tau_cmd output Bus: bus_tau_cmd; bus_tau_ref input Bus: bus_tau_ref; bus_pos_ref input Bus: bus_pos_ref; bus_vel_ref input Bus: bus_vel_ref; bus_kp_kd_dyn input Bus: bus_kp_kd_dyn; bus_pos_state input Bus: bus_pos_state; bus_vel_state input Bus: bus_vel_state; P_G1_CONSTRAINTS parameter
 function bus_tau_cmd = low_level_pd_controller_function( ...
    bus_tau_ref, bus_pos_ref, bus_vel_ref, bus_kp_kd_dyn, ...
    bus_pos_state, bus_vel_state, P_G1_CONSTRAINTS)
%#codegen

% Default output bus
bus_tau_cmd = struct( ...
    'left_hip_pitch',      0, ...
    'left_hip_roll',       0, ...
    'left_hip_yaw',        0, ...
    'left_knee',           0, ...
    'left_ankle_pitch',    0, ...
    'left_ankle_roll',     0, ...
    'right_hip_pitch',     0, ...
    'right_hip_roll',      0, ...
    'right_hip_yaw',       0, ...
    'right_knee',          0, ...
    'right_ankle_pitch',   0, ...
    'right_ankle_roll',    0, ...
    'waist_yaw',           0, ...
    'waist_roll',          0, ...
    'waist_pitch',         0, ...
    'left_shoulder_pitch', 0, ...
    'left_shoulder_roll',  0, ...
    'left_shoulder_yaw',   0, ...
    'left_elbow',          0, ...
    'left_wrist_roll',     0, ...
    'left_wrist_pitch',    0, ...
    'left_wrist_yaw',      0, ...
    'right_shoulder_pitch',0, ...
    'right_shoulder_roll', 0, ...
    'right_shoulder_yaw',  0, ...
    'right_elbow',         0, ...
    'right_wrist_roll',    0, ...
    'right_wrist_pitch',   0, ...
    'right_wrist_yaw',     0, ...
    'left_hand_thumb_0',   0, ...
    'left_hand_thumb_1',   0, ...
    'left_hand_thumb_2',   0, ...
    'left_hand_middle_0',  0, ...
    'left_hand_middle_1',  0, ...
    'left_hand_index_0',   0, ...
    'left_hand_index_1',   0, ...
    'right_hand_thumb_0',  0, ...
    'right_hand_thumb_1',  0, ...
    'right_hand_thumb_2',  0, ...
    'right_hand_middle_0', 0, ...
    'right_hand_middle_1', 0, ...
    'right_hand_index_0',  0, ...
    'right_hand_index_1',  0);

% Unpack reference buses

% tau refs
left_leg_tau_ref   = bus_tau_ref.left_leg_tau_ref;
right_leg_tau_ref  = bus_tau_ref.right_leg_tau_ref;
waist_tau_ref      = bus_tau_ref.waist_tau_ref;
left_arm_tau_ref   = bus_tau_ref.left_arm_tau_ref;
right_arm_tau_ref  = bus_tau_ref.right_arm_tau_ref;

% pos refs
left_leg_pos_ref   = bus_pos_ref.left_leg_pos_ref;
right_leg_pos_ref  = bus_pos_ref.right_leg_pos_ref;
waist_pos_ref      = bus_pos_ref.waist_pos_ref;
left_arm_pos_ref   = bus_pos_ref.left_arm_pos_ref;
right_arm_pos_ref  = bus_pos_ref.right_arm_pos_ref;

% vel refs
left_leg_vel_ref   = bus_vel_ref.left_leg_vel_ref;
right_leg_vel_ref  = bus_vel_ref.right_leg_vel_ref;
waist_vel_ref      = bus_vel_ref.waist_vel_ref;
left_arm_vel_ref   = bus_vel_ref.left_arm_vel_ref;
right_arm_vel_ref  = bus_vel_ref.right_arm_vel_ref;

% dynamic gains
left_leg_kp_kd   = bus_kp_kd_dyn.left_leg_kp_kd_dyn;
right_leg_kp_kd  = bus_kp_kd_dyn.right_leg_kp_kd_dyn;
waist_kp_kd      = bus_kp_kd_dyn.waist_kp_kd_dyn;
left_arm_kp_kd   = bus_kp_kd_dyn.left_arm_kp_kd_dyn;
right_arm_kp_kd  = bus_kp_kd_dyn.right_arm_kp_kd_dyn;

% Unpack state buses

% measured positions
left_leg_pos_state   = bus_pos_state.left_leg_pos_state;
right_leg_pos_state  = bus_pos_state.right_leg_pos_state;
waist_pos_state      = bus_pos_state.waist_pos_state;
left_arm_pos_state   = bus_pos_state.left_arm_pos_state;
right_arm_pos_state  = bus_pos_state.right_arm_pos_state;

% measured velocities
left_leg_vel_state   = bus_vel_state.left_leg_vel_state;
right_leg_vel_state  = bus_vel_state.right_leg_vel_state;
waist_vel_state      = bus_vel_state.waist_vel_state;
left_arm_vel_state   = bus_vel_state.left_arm_vel_state;
right_arm_vel_state  = bus_vel_state.right_arm_vel_state;

% Split Kp / Kd

Kp_left_leg   = left_leg_kp_kd(:,1);
Kd_left_leg   = left_leg_kp_kd(:,2);

Kp_right_leg  = right_leg_kp_kd(:,1);
Kd_right_leg  = right_leg_kp_kd(:,2);

Kp_waist      = waist_kp_kd(:,1);
Kd_waist      = waist_kp_kd(:,2);

Kp_left_arm   = left_arm_kp_kd(:,1);
Kd_left_arm   = left_arm_kp_kd(:,2);

Kp_right_arm  = right_arm_kp_kd(:,1);
Kd_right_arm  = right_arm_kp_kd(:,2);

% Position and velocity errors

e_left_leg   = left_leg_pos_ref   - left_leg_pos_state;
de_left_leg  = left_leg_vel_ref   - left_leg_vel_state;

e_right_leg  = right_leg_pos_ref  - right_leg_pos_state;
de_right_leg = right_leg_vel_ref  - right_leg_vel_state;

e_waist      = waist_pos_ref      - waist_pos_state;
de_waist     = waist_vel_ref      - waist_vel_state;

e_left_arm   = left_arm_pos_ref   - left_arm_pos_state;
de_left_arm  = left_arm_vel_ref   - left_arm_vel_state;

e_right_arm  = right_arm_pos_ref  - right_arm_pos_state;
de_right_arm = right_arm_vel_ref  - right_arm_vel_state;

% PD + feedforward torque
left_leg_tau_cmd   = left_leg_tau_ref   + Kp_left_leg   .* e_left_leg   + Kd_left_leg   .* de_left_leg;
right_leg_tau_cmd  = right_leg_tau_ref  + Kp_right_leg  .* e_right_leg  + Kd_right_leg  .* de_right_leg;
waist_tau_cmd      = waist_tau_ref      + Kp_waist      .* e_waist      + Kd_waist      .* de_waist;
left_arm_tau_cmd   = left_arm_tau_ref   + Kp_left_arm   .* e_left_arm   + Kd_left_arm   .* de_left_arm;
right_arm_tau_cmd  = right_arm_tau_ref  + Kp_right_arm  .* e_right_arm  + Kd_right_arm  .* de_right_arm;

% Torque saturation using robot constraints

tau_abs = P_G1_CONSTRAINTS.tau_abs;

tau_abs_left_leg   = tau_abs(P_G1_CONSTRAINTS.idx_left_leg);
tau_abs_right_leg  = tau_abs(P_G1_CONSTRAINTS.idx_right_leg);
tau_abs_waist      = tau_abs(P_G1_CONSTRAINTS.idx_waist);
tau_abs_left_arm   = tau_abs(P_G1_CONSTRAINTS.idx_left_arm);
tau_abs_right_arm  = tau_abs(P_G1_CONSTRAINTS.idx_right_arm);

left_leg_tau_cmd   = min(max(left_leg_tau_cmd,   -tau_abs_left_leg),   tau_abs_left_leg);
right_leg_tau_cmd  = min(max(right_leg_tau_cmd,  -tau_abs_right_leg),  tau_abs_right_leg);
waist_tau_cmd      = min(max(waist_tau_cmd,      -tau_abs_waist),      tau_abs_waist);
left_arm_tau_cmd   = min(max(left_arm_tau_cmd,   -tau_abs_left_arm),   tau_abs_left_arm);
right_arm_tau_cmd  = min(max(right_arm_tau_cmd,  -tau_abs_right_arm),  tau_abs_right_arm);

% Pack final joint-ordered output bus

% left leg
bus_tau_cmd.left_hip_pitch    = left_leg_tau_cmd(1);
bus_tau_cmd.left_hip_roll     = left_leg_tau_cmd(2);
bus_tau_cmd.left_hip_yaw      = left_leg_tau_cmd(3);
bus_tau_cmd.left_knee         = left_leg_tau_cmd(4);
bus_tau_cmd.left_ankle_pitch  = left_leg_tau_cmd(5);
bus_tau_cmd.left_ankle_roll   = left_leg_tau_cmd(6);

% right leg
bus_tau_cmd.right_hip_pitch   = right_leg_tau_cmd(1);
bus_tau_cmd.right_hip_roll    = right_leg_tau_cmd(2);
bus_tau_cmd.right_hip_yaw     = right_leg_tau_cmd(3);
bus_tau_cmd.right_knee        = right_leg_tau_cmd(4);
bus_tau_cmd.right_ankle_pitch = right_leg_tau_cmd(5);
bus_tau_cmd.right_ankle_roll  = right_leg_tau_cmd(6);

% waist
bus_tau_cmd.waist_yaw         = waist_tau_cmd(1);
bus_tau_cmd.waist_roll        = waist_tau_cmd(2);
bus_tau_cmd.waist_pitch       = waist_tau_cmd(3);

% left arm
bus_tau_cmd.left_shoulder_pitch = left_arm_tau_cmd(1);
bus_tau_cmd.left_shoulder_roll  = left_arm_tau_cmd(2);
bus_tau_cmd.left_shoulder_yaw   = left_arm_tau_cmd(3);
bus_tau_cmd.left_elbow          = left_arm_tau_cmd(4);
bus_tau_cmd.left_wrist_roll     = left_arm_tau_cmd(5);
bus_tau_cmd.left_wrist_pitch    = left_arm_tau_cmd(6);
bus_tau_cmd.left_wrist_yaw      = left_arm_tau_cmd(7);

% right arm
bus_tau_cmd.right_shoulder_pitch = right_arm_tau_cmd(1);
bus_tau_cmd.right_shoulder_roll  = right_arm_tau_cmd(2);
bus_tau_cmd.right_shoulder_yaw   = right_arm_tau_cmd(3);
bus_tau_cmd.right_elbow          = right_arm_tau_cmd(4);
bus_tau_cmd.right_wrist_roll     = right_arm_tau_cmd(5);
bus_tau_cmd.right_wrist_pitch    = right_arm_tau_cmd(6);
bus_tau_cmd.right_wrist_yaw      = right_arm_tau_cmd(7);

% hands disabled for now
bus_tau_cmd.left_hand_thumb_0   = 0;
bus_tau_cmd.left_hand_thumb_1   = 0;
bus_tau_cmd.left_hand_thumb_2   = 0;
bus_tau_cmd.left_hand_middle_0  = 0;
bus_tau_cmd.left_hand_middle_1  = 0;
bus_tau_cmd.left_hand_index_0   = 0;
bus_tau_cmd.left_hand_index_1   = 0;

bus_tau_cmd.right_hand_thumb_0  = 0;
bus_tau_cmd.right_hand_thumb_1  = 0;
bus_tau_cmd.right_hand_thumb_2  = 0;
bus_tau_cmd.right_hand_middle_0 = 0;
bus_tau_cmd.right_hand_middle_1 = 0;
bus_tau_cmd.right_hand_index_0  = 0;
bus_tau_cmd.right_hand_index_1  = 0;

end

== matlab function Sim2Real_ankle_motion_2025a/SIM2REAL VARIANT SUBSYSTEM/MuJoCo SUBSYSTEM/MuJoCo SUBSYSTEM/JOINT STATE/IMU GRAPH ==
  settings: updateMethod=DISCRETE
  data: bus_imu input Bus: bus_imu; P_MACHINE_DATA parameter
function imu_graph_function(bus_imu, P_MACHINE_DATA)
%#codegen

coder.extrinsic('figure','subplot','plot3','line','legend','title', ...
                'grid','axis','xlim','ylim','zlim','view','hold','set', ...
                'drawnow','text','xlabel','ylabel');

persistent fig ax3 axA axG ...
           hX hY hZ ...
           la1 la2 la3 ...
           lg1 lg2 lg3 ...
           txtYPR ...
           Tbuf Abuf Gbuf ...
           Nbuf nsamp kbuf ...
           inited ...
           windowSec ...
           Ts_ui ...
           frame_count ...
           orient_div ...
           axis_div ...
           last_xlim_update

if ~(P_MACHINE_DATA.active_IMU_graph ~= 0)
    return;
end

Ts_ui = double(P_MACHINE_DATA.Ts_UIs);
if ~isfinite(Ts_ui) || Ts_ui <= 0
    Ts_ui = 0.05;
end

quat = double(bus_imu.quat(:));   % [w x y z]
gyro = double(bus_imu.gyro(:));   % [rad/s]
acc  = double(bus_imu.acc(:));    % [m/s^2]

if numel(quat) ~= 4 || numel(gyro) ~= 3 || numel(acc) ~= 3
    return;
end

if isempty(inited)
    windowSec = 1.5;
    Nbuf = max(20, ceil(windowSec / Ts_ui) + 3);
    Tbuf = zeros(1, Nbuf);
    Abuf = zeros(3, Nbuf);
    Gbuf = zeros(3, Nbuf);
    nsamp = uint32(0);
    kbuf  = uint32(0);
    frame_count = uint32(0);
    orient_div = uint32(6);   
    axis_div   = uint32(10);  
    last_xlim_update = 0.0;
    fig = figure('Name','IMU State','Position',[80 80 900 900], 'Tag','G1_IMUState');
    ax3 = subplot(3,1,1,'Parent',fig);
    title(ax3, {'IMU frame [quat]'; ' '});
    grid(ax3,'on');
    axis(ax3,'equal');
    xlim(ax3,[-1.1 1.1]);
    ylim(ax3,[-1.1 1.1]);
    zlim(ax3,[-1.1 1.1]);
    view(ax3,55,25);
    hold(ax3,'on');
    plot3(ax3,[-1.1 1.1],[0 0],[0 0],'k:');
    plot3(ax3,[0 0],[-1.1 1.1],[0 0],'k:');
    plot3(ax3,[0 0],[0 0],[-1.1 1.1],'k:');
    hX = plot3(ax3,[0 1],[0 0],[0 0],'LineWidth',3,'Color',[1 0 0]);
    hY = plot3(ax3,[0 0],[0 1],[0 0],'LineWidth',3,'Color',[0 0.5 0]);
    hZ = plot3(ax3,[0 0],[0 0],[0 1],'LineWidth',3,'Color',[0 0 1]);
    text(ax3, 1.675, 0.75, ' IMU frame [RPY]', ...
        'Units','normalized', ...
        'HorizontalAlignment','left', ...
        'FontWeight','bold', ...
        'FontSize',10, ...
        'Clipping','off');
    txtYPR = text(ax3, 1.675, 0.50, ...
        sprintf(['\\color[rgb]{1,0,0}Roll:  %+.2f°\\color{black}\n' ...
         '\\color[rgb]{0,0.5,0}Pitch: %+.2f°\\color{black}\n' ...
         '\\color[rgb]{0,0,1}Yaw:   %+.2f°\\color{black}'],0,0,0), ...
        'Units','normalized', ...
        'HorizontalAlignment','left', ...
        'Interpreter','tex', ...
        'FontWeight','bold', ...
        'BackgroundColor','none', ...
        'Color','k', ...
        'FontName','FixedWidth', ...
        'FontSize',11, ...
        'Clipping','off');
    hold(ax3,'off');
    set(ax3,'Position',[0.05 0.68 0.60 0.25]);

    axA = subplot(3,1,2,'Parent',fig);
    grid(axA,'on');
    title(axA,'Accelerometer');
    ylabel(axA,'Amplitude [m/s^2]');
    xlabel(axA,'Time [s]');
    xlim(axA,[-windowSec 0.0]);
    la1 = line(axA,0,0,'Color',[1 0 0]);
    la2 = line(axA,0,0,'Color',[0 0.5 0]);
    la3 = line(axA,0,0,'Color',[0 0 1]);
    legend(axA,{'ax','ay','az'},'Location','northeastoutside');

    axG = subplot(3,1,3,'Parent',fig);
    grid(axG,'on');
    title(axG,'Gyro');
    xlabel(axG,'Time [s]');
    ylabel(axG,'Amplitude [rad/s]');
    xlim(axG,[-windowSec 0.0]);
    lg1 = line(axG,0,0,'Color',[1 0 0]);
    lg2 = line(axG,0,0,'Color',[0 0.5 0]);
    lg3 = line(axG,0,0,'Color',[0 0 1]);
    legend(axG,{'gx','gy','gz'},'Location','northeastoutside');
    inited = true;
end

kbuf = kbuf + uint32(1);
if kbuf > uint32(Nbuf)
    kbuf = uint32(1);
end
k = double(kbuf);
if nsamp < uint32(Nbuf)
    nsamp = nsamp + uint32(1);
end
n = double(nsamp);
frame_count = frame_count + uint32(1);
if n == 1
    Tbuf(1,k) = 0.0;
else
    if k == 1
        kprev = Nbuf;
    else
        kprev = k - 1;
    end
    Tbuf(1,k) = Tbuf(1,kprev) + Ts_ui;
end
Abuf(:,k) = -acc(:);
Gbuf(:,k) = gyro(:);

if n < Nbuf
    tt = Tbuf(1,1:n);
    aa = Abuf(:,1:n);
    gg = Gbuf(:,1:n);
else
    if k < Nbuf
        ord = [k+1:Nbuf, 1:k];
    else
        ord = 1:Nbuf;
    end
    tt = Tbuf(ord);
    aa = Abuf(:,ord);
    gg = Gbuf(:,ord);
end

if ~isempty(tt)
    tt = tt - tt(end);
end

if mod(double(frame_count), double(orient_div)) == 0
    R  = quat2rotm_wxyz(quat(:)');
    ex = R(:,1);
    ey = R(:,2);
    ez = R(:,3);
    set(hX,'XData',[0 ex(1)],'YData',[0 ex(2)],'ZData',[0 ex(3)]);
    set(hY,'XData',[0 ey(1)],'YData',[0 ey(2)],'ZData',[0 ey(3)]);
    set(hZ,'XData',[0 ez(1)],'YData',[0 ez(2)],'ZData',[0 ez(3)]);
    [yaw,pitch,roll] = quat_to_ypr_zyx(quat(:)');
    set(txtYPR,'String',sprintf([ ...
        '\\color[rgb]{1,0,0}Roll:  %+.2f°\\color{black}\n' ...
        '\\color[rgb]{0,0.5,0}Pitch: %+.2f°\\color{black}\n' ...
        '\\color[rgb]{0,0,1}Yaw:   %+.2f°\\color{black}'], ...
        roll*180/pi, pitch*180/pi, yaw*180/pi));
end

set(la1,'XData',tt,'YData',aa(1,:));
set(la2,'XData',tt,'YData',aa(2,:));
set(la3,'XData',tt,'YData',aa(3,:));
set(lg1,'XData',tt,'YData',gg(1,:));
set(lg2,'XData',tt,'YData',gg(2,:));
set(lg3,'XData',tt,'YData',gg(3,:));

if mod(double(frame_count), double(axis_div)) == 0
    if abs(last_xlim_update - tt(end)) > 0.25 || frame_count == uint32(1)
        xlim(axA,[-windowSec 0.0]);
        xlim(axG,[-windowSec 0.0]);
        last_xlim_update = tt(end);
    end
    ylim_soft_fast(axA, aa);
    ylim_soft_fast(axG, gg);
end
drawnow limitrate nocallbacks;
end

function R = quat2rotm_wxyz(q)
w=q(1); x=q(2); y=q(3); z=q(4);
xx=x*x; yy=y*y; zz=z*z; wx=w*x; wy=w*y; wz=w*z; xy=x*y; xz=x*z; yz=y*z;
R=[1-2*(yy+zz)  2*(xy-wz)  2*(xz+wy);
   2*(xy+wz)  1-2*(xx+zz)  2*(yz-wx);
   2*(xz-wy)  2*(yz+wx)    1-2*(xx+yy)];
end

function [yaw,pitch,roll] = quat_to_ypr_zyx(q)
w=q(1); x=q(2); y=q(3); z=q(4);
yaw   = atan2(2*(w*z + x*y), 1 - 2*(y*y + z*z));
pitch = asin(max(-1,min(1, 2*(w*y - z*x))));
roll  = atan2(2*(w*x + y*z), 1 - 2*(x*x + y*y));
end

function ylim_soft_fast(ax, Y)
if isempty(Y)
    ylim(ax,[-1 1]);
    return;
end

m1 = max(abs(Y(1,:)));
m2 = max(abs(Y(2,:)));
m3 = max(abs(Y(3,:)));
v = max(1e-6, max([m1 m2 m3]));
ylim(ax,[-1.2*v, 1.2*v]);
end

== matlab function Sim2Real_ankle_motion_2025a/KP KD LOW LEVEL - PD ==
  data: enable_gains input; bus_out output Bus: bus_kp_kd_dyn
function bus_out = kp_kd_constants(enable_gains)
%#codegen

    % LEGS: [Kp Kd]
    KP_KD_ANKLE_PITCH = [60 2];
    KP_KD_ANKLE_ROLL  = [60 2];

    bus_out.left_leg_kp_kd_dyn  = zeros(6,2);
    bus_out.right_leg_kp_kd_dyn = zeros(6,2);
    bus_out.waist_kp_kd_dyn     = zeros(3,2);
    bus_out.left_arm_kp_kd_dyn  = zeros(7,2);
    bus_out.right_arm_kp_kd_dyn = zeros(7,2);

    if enable_gains ~= 0
        bus_out.left_leg_kp_kd_dyn(5,:) = KP_KD_ANKLE_PITCH;
        bus_out.left_leg_kp_kd_dyn(6,:) = KP_KD_ANKLE_ROLL;
        bus_out.right_leg_kp_kd_dyn(5,:) = KP_KD_ANKLE_PITCH;
        bus_out.right_leg_kp_kd_dyn(6,:) = KP_KD_ANKLE_ROLL;
    end
end
